simulink model "sim_config2a"  (R2023b)
settings: Solver=ode4  StartTime=0.0  StopTime=60  FixedStep=0.01  RelTol=1e-3
undefined symbols (not defined in the file): aircraft, alt_ground, atmosphere, envir, g, pos_ref, struct2cell, u0, wind
libraries: unit_conversions_lib x19, flightgear_visualization_lib x2, joystick_lib x1, atmosphere_lib x1, axes_transformation_lib x1, syntrac_lib x1
settings Model: Creator=yannic  LastModifiedBy=Ole Bunde

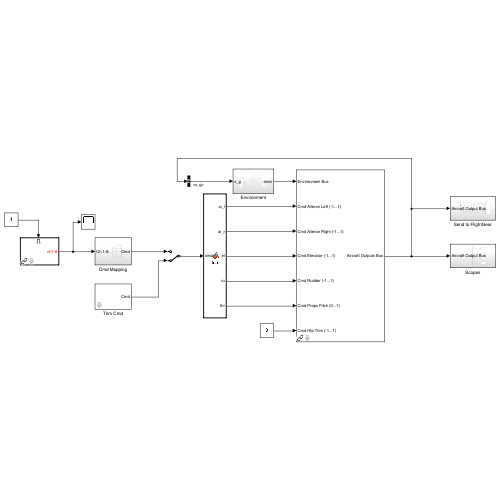
[thumbnail: Simulink's stored preview of the top-level diagram]
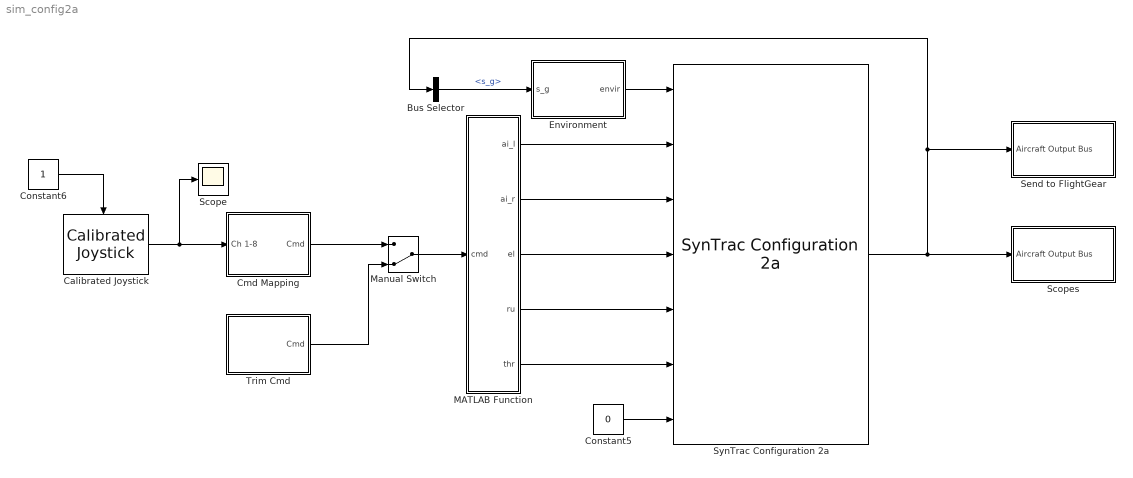
== system sim_config2a ==
  Bus Selector : BusSelector  OutputSignals=rigidBodyBus.s_g
  Calibrated Joystick : joystick_lib/Calibrated Joystick  jystck=jystck  joyid=1
      settings: SourceProductName=LADAC
  Cmd Mapping : Subsystem
  Constant5 : Constant  Value=0
  Constant6 : Constant
  Environment : Subsystem
  MATLAB Function : MATLAB Function  TreatAsAtomicUnit=on
  Manual Switch : ManualSwitch  CurrentSetting=0
  Scope : Scope
  Scopes : Subsystem
  Send to FlightGear : Subsystem
  SynTrac Configuration 2a : syntrac_lib/SynTrac Configuration 2a  aircraft=aircraft  ic=ic
  Trim Cmd : Subsystem  mask{num_props=length(aircraft.prop)}
      mask prompts: num_props "Number of Propellers"
  wires:
  Environment/1(envir) -> SynTrac Configuration 2a/1
  SynTrac Configuration 2a/1 -> Send to FlightGear/1(Aircraft Output Bus), Bus Selector/1, Scopes/1(Aircraft Output Bus)
  Bus Selector/1 -> Environment/1(s_g)  "<s_g>"
  Constant5/1 -> SynTrac Configuration 2a/7
  Constant6/1 -> Calibrated Joystick/Enable
  Calibrated Joystick/1 -> Cmd Mapping/1(Ch 1-8), Scope/1
  Cmd Mapping/1(Cmd) -> Manual Switch/1
  Manual Switch/1 -> MATLAB Function/1(cmd)
  MATLAB Function/5(thr) -> SynTrac Configuration 2a/6
  MATLAB Function/4(ru) -> SynTrac Configuration 2a/5
  MATLAB Function/2(ai_r) -> SynTrac Configuration 2a/3
  MATLAB Function/1(ai_l) -> SynTrac Configuration 2a/2
  Trim Cmd/1(Cmd) -> Manual Switch/2
  MATLAB Function/3(el) -> SynTrac Configuration 2a/4

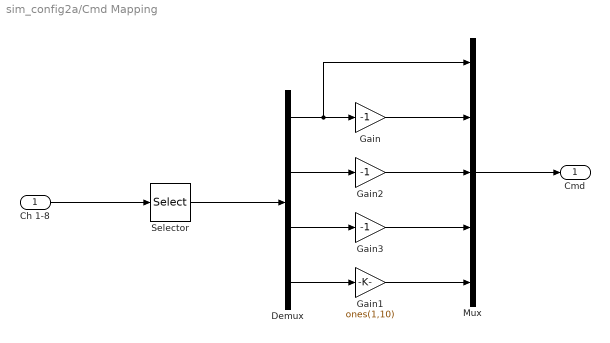
== system sim_config2a/Cmd Mapping ==
  Ch 1-8 : Inport
  Demux : Demux
  Gain : Gain  Gain=-1
  Gain1 : Gain  Gain=ones(1,10)
  Gain2 : Gain  Gain=-1
  Gain3 : Gain  Gain=-1
  Mux : Mux  Inputs=5
  Selector : Selector  InputPortWidth=8  IndexOptions=Index vector (dialog)  Indices=[1,2,3,4]  OutputSizes=1
  Cmd : Outport
  wires:
  Gain1/1 -> Mux/5
  Demux/4 -> Gain1/1
  Gain/1 -> Mux/2
  Gain2/1 -> Mux/3
  Demux/3 -> Gain3/1
  Demux/2 -> Gain2/1
  Demux/1 -> Mux/1, Gain/1
  Ch 1-8/1 -> Selector/1
  Gain3/1 -> Mux/4
  Mux/1 -> Cmd/1
  Selector/1 -> Demux/1

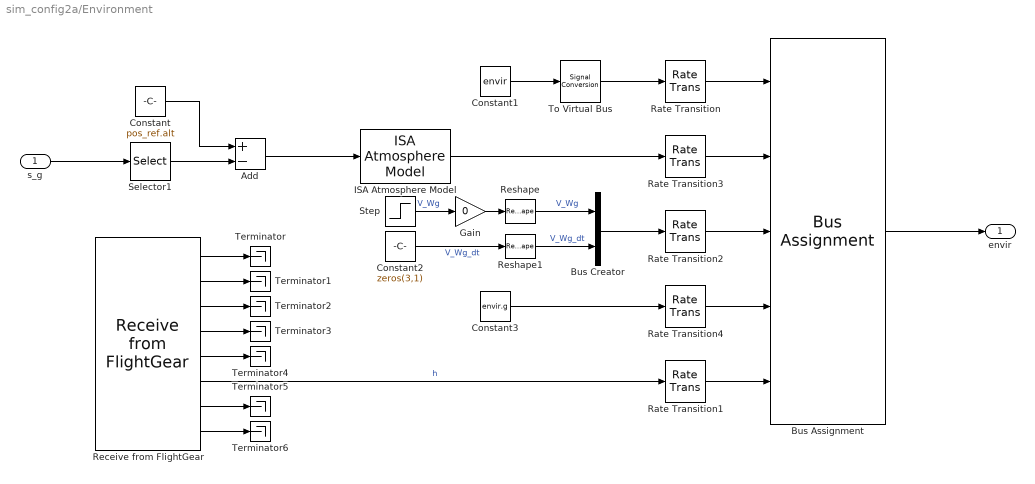
== system sim_config2a/Environment ==
  s_g : Inport
  Add : Sum  Inputs=+-
  Bus Assignment : BusAssignment  AssignedSignals=atmosphere,wind,g,alt_ground
  Bus Creator : BusCreator  Inputs=2
  Constant : Constant  Value=pos_ref.alt
  Constant1 : Constant  Value=envir  OutDataTypeStr=Bus: envirBus
  Constant2 : Constant  Value=zeros(3,1)
  Constant3 : Constant  Value=envir.g
  Gain : Gain  Gain=0
  ISA Atmosphere Model : atmosphere_lib/ISA Atmosphere Model
      settings: SourceProductName=LADAC
  Rate Transition{,1..4} (5 alike) : RateTransition
  Receive from FlightGear : flightgear_visualization_lib/Receive from FlightGear  ip_address='127.0.0.1'  ip_port=5503  sample_time=1/20  blocking_time=0  is_aerocntrl=off  is_engine=off  is_fuel=off  is_land=off  is_avionics=off  is_envir=on
  Reshape : Reshape  OutputDimensionality=Column vector (2-D)
  Reshape1 : Reshape  OutputDimensionality=Column vector (2-D)
  Selector1 : Selector  InputPortWidth=3  IndexOptions=Index vector (dialog)  Indices=3  OutputSizes=1
  Step : Step  Time=3  After=[0;9;0]  SampleTime=0
  Terminator{,1..6} (7 alike) : Terminator
  To Virtual Bus : SignalConversion  ConversionOutput=Virtual bus  OverrideOpt=off
  envir : Outport  VectorParamsAs1DForOutWhenUnconnected=off
  wires:
  Rate Transition2/1 -> Bus Assignment/3
  Rate Transition3/1 -> Bus Assignment/2
  Bus Assignment/1 -> envir/1
  Rate Transition/1 -> Bus Assignment/1
  ISA Atmosphere Model/1 -> Rate Transition3/1
  Step/1 -> Gain/1  "V_Wg"
  Rate Transition1/1 -> Bus Assignment/5
  Constant1/1 -> To Virtual Bus/1
  s_g/1 -> Selector1/1
  Bus Creator/1 -> Rate Transition2/1
  Constant2/1 -> Reshape1/1  "V_Wg_dt"
  Rate Transition4/1 -> Bus Assignment/4
  Constant3/1 -> Rate Transition4/1
  Gain/1 -> Reshape/1
  Constant/1 -> Add/1
  Add/1 -> ISA Atmosphere Model/1
  Selector1/1 -> Add/2
  To Virtual Bus/1 -> Rate Transition/1
  Reshape/1 -> Bus Creator/1  "V_Wg"
  Reshape1/1 -> Bus Creator/2  "V_Wg_dt"
  Receive from FlightGear/3 -> Terminator2/1
  Receive from FlightGear/1 -> Terminator/1
  Receive from FlightGear/6 -> Rate Transition1/1  "h"
  Receive from FlightGear/2 -> Terminator1/1
  Receive from FlightGear/5 -> Terminator4/1
  Receive from FlightGear/7 -> Terminator5/1
  Receive from FlightGear/4 -> Terminator3/1
  Receive from FlightGear/8 -> Terminator6/1

== system sim_config2a/Scopes ==
  Aircraft Output Bus : Inport
  Actuators : Subsystem
  Aerodynamics : Subsystem
  Bus Selector : BusSelector  OutputSignals=rigidBodyBus,aeroBus,actuatorsBus,propBus
  Propellers : Subsystem
  Rigid Body : Subsystem
  wires:
  Aircraft Output Bus/1 -> Bus Selector/1
  Bus Selector/1 -> Rigid Body/1(rigidBodyBus)  "<rigidBodyBus>"
  Bus Selector/3 -> Actuators/1(actuatorsBus)  "<actuatorsBus>"
  Bus Selector/2 -> Aerodynamics/1(aeroBus)  "<aeroBus>"
  Bus Selector/4 -> Propellers/1(propBus)  "<propBus>"

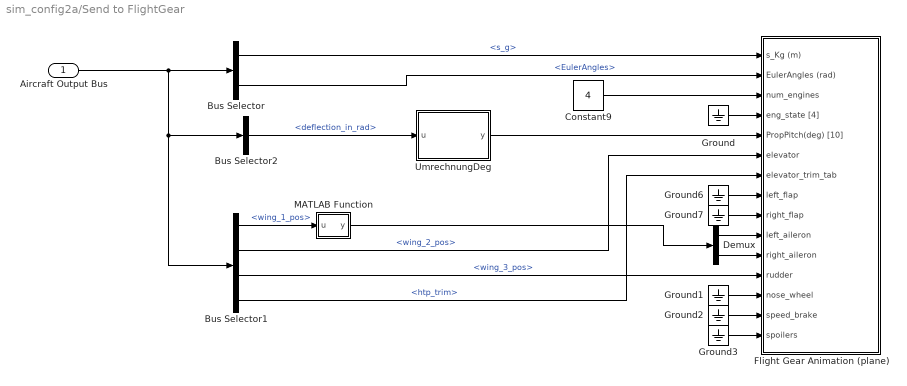
== system sim_config2a/Send to FlightGear ==
  Aircraft Output Bus : Inport
  Bus Selector : BusSelector  OutputSignals=rigidBodyBus.s_g,rigidBodyBus.EulerAngles
  Bus Selector1 : BusSelector  OutputSignals=actuatorsBus.wing_1_pos,actuatorsBus.wing_2_pos,actuatorsBus.wing_3_pos,actuatorsBus.htp_trim
  Bus Selector2 : BusSelector  OutputSignals=actuatorsBus.props_pitch.deflection_in_rad
  Constant9 : Constant  Value=4
  Demux : Demux  Outputs=2
  Flight Gear Animation (plane) : Subsystem  AncestorBlock=flightgear_visualization_lib/Flight Gear Animation (plane)  mask{inital_lat=pos_ref.lat, inital_long=pos_ref.lon, inital_height=pos_ref.alt, remoteURL='127.0.0.1', remotePort=5502}
      mask prompts: inital_lat "Inital Latitude (deg)"; inital_long "Inital Longitude (deg)"; inital_height "Inital Height (m)"; remoteURL "URL of FlightGear, e.g. '127.0.0.1'"; remotePort "Port of FlightGear, e.g. 5502"
      mask TypeOptions remoteURL: Send to FlightGear/remoteURL
      mask TypeOptions remotePort: Send to FlightGear/remotePort
      mask DialogControl GroupDesc Prompt: Initial Latitude
  Ground{,1..3,6..7} (6 alike) : Ground
  MATLAB Function : MATLAB Function  TreatAsAtomicUnit=on
  UmrechnungDeg : MATLAB Function  TreatAsAtomicUnit=on
  wires:
  Bus Selector/1 -> Flight Gear Animation (plane)/1(s_Kg (m))  "<s_g>"
  Bus Selector/2 -> Flight Gear Animation (plane)/2(EulerAngles (rad))  "<EulerAngles>"
  Constant9/1 -> Flight Gear Animation (plane)/3(num_engines)
  Ground/1 -> Flight Gear Animation (plane)/4(eng_state [4])
  Ground1/1 -> Flight Gear Animation (plane)/13(nose_wheel)
  Ground2/1 -> Flight Gear Animation (plane)/14(speed_brake)
  Ground3/1 -> Flight Gear Animation (plane)/15(spoilers)
  Aircraft Output Bus/1 -> Bus Selector1/1, Bus Selector2/1, Bus Selector/1
  Bus Selector1/2 -> Flight Gear Animation (plane)/6(elevator)  "<wing_2_pos>"
  Bus Selector1/4 -> Flight Gear Animation (plane)/7(elevator_trim_tab)  "<htp_trim>"
  Ground6/1 -> Flight Gear Animation (plane)/8(left_flap)
  Ground7/1 -> Flight Gear Animation (plane)/9(right_flap)
  Bus Selector1/3 -> Flight Gear Animation (plane)/12(rudder)  "<wing_3_pos>"
  Bus Selector1/1 -> MATLAB Function/1(u)  "<wing_1_pos>"
  Demux/1 -> Flight Gear Animation (plane)/10(left_aileron)
  Demux/2 -> Flight Gear Animation (plane)/11(right_aileron)
  MATLAB Function/1(y) -> Demux/1
  Bus Selector2/1 -> UmrechnungDeg/1(u)  "<deflection_in_rad>"
  UmrechnungDeg/1(y) -> Flight Gear Animation (plane)/5(PropPitch(deg) [10])

== system sim_config2a/Trim Cmd ==
  u0 : Constant  Value=cell2mat(struct2cell(u0))
  u0 to Cmd : MATLAB Function  TreatAsAtomicUnit=on
  Cmd : Outport
  wires:
  u0/1 -> u0 to Cmd/1(u0)
  u0 to Cmd/1(cmd) -> Cmd/1

== system sim_config2a/Scopes/Actuators ==
  actuatorsBus : Inport
  Aileron Deflections (deg) (Downward Positive) : Scope
  Bus Selector : BusSelector  OutputSignals=wing_1_pos,wing_2_pos,wing_3_pos,props_pitch.deflection_in_rad,htp_trim
  Elevator Deflection (deg) (Downward Positive) : Scope
  Propeller Pitch (deg) : Scope
  Rudder Deflection (deg) (Right Positive) : Scope
  Scope : Scope
  rad2deg : unit_conversions_lib/rad2deg
      settings: SourceProductName=LADAC
  wires:
  actuatorsBus/1 -> Bus Selector/1
  Bus Selector/1 -> Aileron Deflections (deg) (Downward Positive)/1  "<wing_1_pos>"
  Bus Selector/2 -> Elevator Deflection (deg) (Downward Positive)/1  "<wing_2_pos>"
  Bus Selector/3 -> Rudder Deflection (deg) (Right Positive)/1  "<wing_3_pos>"
  Bus Selector/4 -> rad2deg/1  "<deflection_in_rad>"
  rad2deg/1 -> Propeller Pitch (deg)/1
  Bus Selector/5 -> Scope/1  "<htp_trim>"

== system sim_config2a/Scopes/Aerodynamics ==
  aeroBus : Inport
  Bus Selector : BusSelector  OutputSignals=main,htp,vtp,R_Ab,Q_Ab
  Force Vector (N) (Body Frame) : Scope
  Horizontal Tailplane : Subsystem
  Main Wing : Subsystem
  Moment Vector (Nm) (Body Frame) : Scope
  Vertical Tailplane : Subsystem
  wires:
  aeroBus/1 -> Bus Selector/1
  Bus Selector/1 -> Main Wing/1(wingBus)  "<main>"
  Bus Selector/2 -> Horizontal Tailplane/1(wingBus)  "<htp>"
  Bus Selector/3 -> Vertical Tailplane/1(wingBus)  "<vtp>"
  Bus Selector/4 -> Force Vector (N) (Body Frame)/1  "<R_Ab>"
  Bus Selector/5 -> Moment Vector (Nm) (Body Frame)/1  "<Q_Ab>"

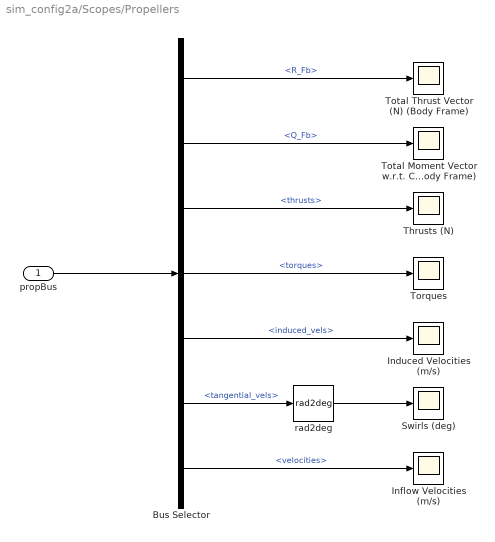
== system sim_config2a/Scopes/Propellers ==
  propBus : Inport
  Bus Selector : BusSelector  OutputSignals=R_Fb,Q_Fb,thrusts,torques,induced_vels,tangential_vels,velocities
  Induced Velocities (m/s) : Scope
  Inflow Velocities (m/s) : Scope
  Swirls (deg) : Scope
  Thrusts (N) : Scope
  Torques : Scope
  Total Moment Vector w.r.t. CG (Nm) (Body Frame) : Scope
  Total Thrust Vector (N) (Body Frame) : Scope
  rad2deg : unit_conversions_lib/rad2deg
      settings: SourceProductName=LADAC
  wires:
  propBus/1 -> Bus Selector/1
  Bus Selector/1 -> Total Thrust Vector (N) (Body Frame)/1  "<R_Fb>"
  Bus Selector/2 -> Total Moment Vector w.r.t. CG (Nm) (Body Frame)/1  "<Q_Fb>"
  Bus Selector/3 -> Thrusts (N)/1  "<thrusts>"
  Bus Selector/4 -> Torques/1  "<torques>"
  Bus Selector/5 -> Induced Velocities (m/s)/1  "<induced_vels>"
  Bus Selector/6 -> rad2deg/1  "<tangential_vels>"
  rad2deg/1 -> Swirls (deg)/1
  Bus Selector/7 -> Inflow Velocities (m/s)/1  "<velocities>"

== system sim_config2a/Scopes/Rigid Body ==
  rigidBodyBus : Inport
  Angular Rates (deg/s) : Scope
  Bus Selector : BusSelector  OutputSignals=omega_Kb,EulerAngles,s_g,V_Kg,V_Kb
  Euler Angles (deg) : Scope
  Position (m) : Scope
  Velocity FRD (m/s) : Scope
  Velocity NED (m/s) : Scope
  rad2deg : unit_conversions_lib/rad2deg
      settings: SourceProductName=LADAC
  rad2deg1 : unit_conversions_lib/rad2deg
      settings: SourceProductName=LADAC
  wires:
  rigidBodyBus/1 -> Bus Selector/1
  Bus Selector/1 -> rad2deg/1  "<omega_Kb>"
  rad2deg/1 -> Angular Rates (deg/s)/1
  Bus Selector/2 -> rad2deg1/1  "<EulerAngles>"
  rad2deg1/1 -> Euler Angles (deg)/1
  Bus Selector/3 -> Position (m)/1  "<s_g>"
  Bus Selector/4 -> Velocity NED (m/s)/1  "<V_Kg>"
  Bus Selector/5 -> Velocity FRD (m/s)/1  "<V_Kb>"

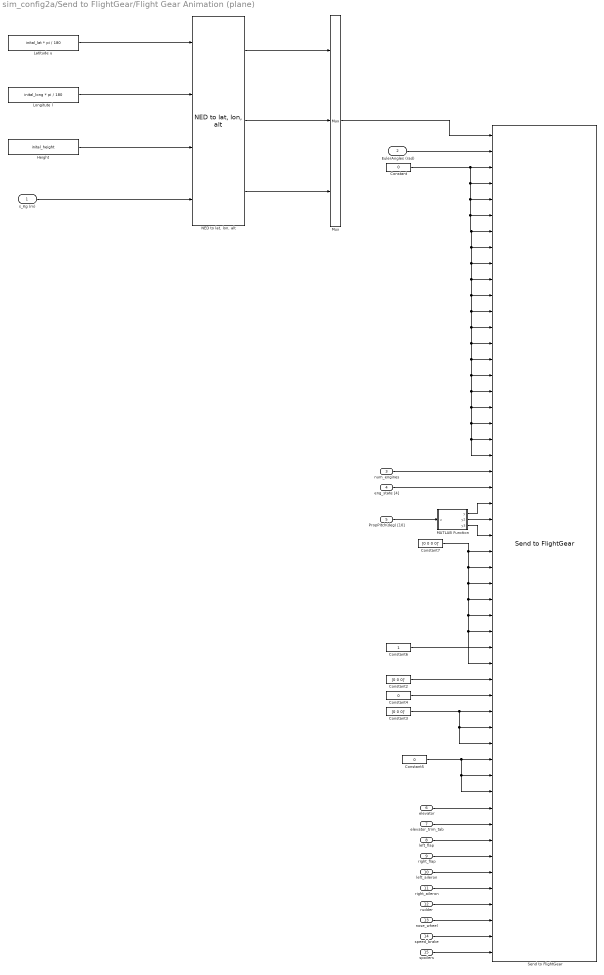
== system sim_config2a/Send to FlightGear/Flight Gear Animation (plane) ==
  s_Kg (m) : Inport
  EulerAngles (rad) : Inport  Port=2
  num_engines : Inport  Port=3  PortDimensions=[1]
  eng_state [4] : Inport  Port=4  PortDimensions=[4]
  PropPitch(deg) [10] : Inport  Port=5  PortDimensions=[10]
  elevator : Inport  Port=6  PortDimensions=[1]
  elevator_trim_tab : Inport  Port=7  PortDimensions=[1]
  left_flap : Inport  Port=8  PortDimensions=[1]
  right_flap : Inport  Port=9  PortDimensions=[1]
  left_aileron : Inport  Port=10  PortDimensions=[1]
  right_aileron : Inport  Port=11  PortDimensions=[1]
  rudder : Inport  Port=12  PortDimensions=[1]
  nose_wheel : Inport  Port=13  PortDimensions=[1]
  speed_brake : Inport  Port=14  PortDimensions=[1]
  spoilers : Inport  Port=15  PortDimensions=[1]
  Constant : Constant  Value=0
  Constant2 : Constant  Value=[0 0 0]'  VectorParams1D=off
  Constant3 : Constant  Value=[0 0 0]'  VectorParams1D=off
  Constant4 : Constant  Value=0
  Constant5 : Constant  Value=0
  Constant6 : Constant
  Constant7 : Constant  Value=[0 0 0 0]'  VectorParams1D=off
  Height : Constant  Value=inital_height
  Latitude u : Constant  Value=inital_lat * pi / 180
  Longitute l : Constant  Value=inital_long * pi / 180
  MATLAB Function : MATLAB Function  TreatAsAtomicUnit=on
  Mux : Mux  Inputs=3
  "NED to lat, lon, alt" : axes_transformation_lib/NED to lat, lon, alt  SystemSampleTime=-1  VariantActivationTime=update diagram  AllowFlexibleInterface=on  Latency=0  AutoFrameSizeCalculation=off
      settings: SourceProductName=LADAC
  Send to FlightGear : flightgear_visualization_lib/Send to FlightGear  remotePort=remotePort  remoteURL=remoteURL
  wires:
  Constant6/1 -> Send to FlightGear/33
  Constant5/1 -> Send to FlightGear/41, Send to FlightGear/42, Send to FlightGear/40
  Constant4/1 -> Send to FlightGear/36
  Constant3/1 -> Send to FlightGear/38, Send to FlightGear/39, Send to FlightGear/37
  Constant2/1 -> Send to FlightGear/35
  Constant7/1 -> Send to FlightGear/34, Send to FlightGear/32, Send to FlightGear/31, Send to FlightGear/30, Send to FlightGear/29, Send to FlightGear/28, Send to FlightGear/27
  Constant/1 -> Send to FlightGear/20, Send to FlightGear/21, Send to FlightGear/19, Send to FlightGear/18, Send to FlightGear/17, Send to FlightGear/16, Send to FlightGear/15, Send to FlightGear/14, Send to FlightGear/13, Send to FlightGear/12, Send to FlightGear/11, Send to FlightGear/10, Send to FlightGear/9, Send to FlightGear/8, Send to FlightGear/7, Send to FlightGear/6, Send to FlightGear/5, Send to FlightGear/4, Send to FlightGear/3
  PropPitch(deg) [10]/1 -> MATLAB Function/1(u)
  eng_state [4]/1 -> Send to FlightGear/23
  num_engines/1 -> Send to FlightGear/22
  right_aileron/1 -> Send to FlightGear/48
  left_aileron/1 -> Send to FlightGear/47
  right_flap/1 -> Send to FlightGear/46
  left_flap/1 -> Send to FlightGear/45
  elevator_trim_tab/1 -> Send to FlightGear/44
  elevator/1 -> Send to FlightGear/43
  rudder/1 -> Send to FlightGear/49
  nose_wheel/1 -> Send to FlightGear/50
  speed_brake/1 -> Send to FlightGear/51
  spoilers/1 -> Send to FlightGear/52
  s_Kg (m)/1 -> "NED to lat, lon, alt"/4
  EulerAngles (rad)/1 -> Send to FlightGear/2
  Latitude u/1 -> "NED to lat, lon, alt"/1
  Longitute l/1 -> "NED to lat, lon, alt"/2
  Height/1 -> "NED to lat, lon, alt"/3
  "NED to lat, lon, alt"/3 -> Mux/3
  "NED to lat, lon, alt"/2 -> Mux/2
  "NED to lat, lon, alt"/1 -> Mux/1
  Mux/1 -> Send to FlightGear/1
  MATLAB Function/1(y) -> Send to FlightGear/24
  MATLAB Function/2(y2) -> Send to FlightGear/25
  MATLAB Function/3(y3) -> Send to FlightGear/26

== system sim_config2a/Scopes/Aerodynamics/Horizontal Tailplane ==
  wingBus : Inport
  Aerodynamics : Subsystem
  Body : Subsystem
  Bus Selector : BusSelector  OutputSignals=body,aero,external.V_Wb
  Wind/Slipstream : Subsystem
  wires:
  Bus Selector/3 -> Wind/Slipstream/1(V_Wb)  "<V_Wb>"
  Bus Selector/2 -> Aerodynamics/1(aeroBus)  "<aero>"
  Bus Selector/1 -> Body/1(bodyBus)  "<body>"
  wingBus/1 -> Bus Selector/1

== system sim_config2a/Scopes/Aerodynamics/Main Wing ==
  wingBus : Inport
  Aerodynamics : Subsystem
  Body : Subsystem
  Bus Selector : BusSelector  OutputSignals=body,aero,external.V_Wb
  Wind/Slipstream : Subsystem
  wires:
  wingBus/1 -> Bus Selector/1
  Bus Selector/1 -> Body/1(bodyBus)  "<body>"
  Bus Selector/2 -> Aerodynamics/1(aeroBus)  "<aero>"
  Bus Selector/3 -> Wind/Slipstream/1(V_Wb)  "<V_Wb>"

== system sim_config2a/Scopes/Aerodynamics/Vertical Tailplane ==
  wingBus : Inport
  Aerodynamics : Subsystem
  Body : Subsystem
  Bus Selector : BusSelector  OutputSignals=body,aero,external.V_Wb
  Wind/Slipstream : Subsystem
  wires:
  wingBus/1 -> Bus Selector/1
  Bus Selector/1 -> Body/1(bodyBus)  "<body>"
  Bus Selector/2 -> Aerodynamics/1(aeroBus)  "<aero>"
  Bus Selector/3 -> Wind/Slipstream/1(V_Wb)  "<V_Wb>"

== system sim_config2a/Scopes/Aerodynamics/Horizontal Tailplane/Aerodynamics ==
  aeroBus : Inport
  Bus Selector : BusSelector  OutputSignals=circulation,coeff_loc,coeff_glob,force_loc,force_glob,local_inflow
  Circulation : Subsystem
  Global Coefficients : Subsystem
  Global Forces : Subsystem
  Local Coefficients : Subsystem
  Local Forces : Subsystem
  Local Inflow : Subsystem
  wires:
  Bus Selector/6 -> Local Inflow/1(localInflowBus)  "<local_inflow>"
  Bus Selector/5 -> Global Forces/1(forceGlobBus)  "<force_glob>"
  Bus Selector/4 -> Local Forces/1(forceLocBus)  "<force_loc>"
  Bus Selector/3 -> Global Coefficients/1(coeffGlobBus)  "<coeff_glob>"
  aeroBus/1 -> Bus Selector/1
  Bus Selector/1 -> Circulation/1(circulationBus)  "<circulation>"
  Bus Selector/2 -> Local Coefficients/1(coeffLocBus)  "<coeff_loc>"

== system sim_config2a/Scopes/Aerodynamics/Horizontal Tailplane/Body ==
  bodyBus : Inport
  Airspeed (m/s) : Scope
  Angle of Attack (deg) : Scope
  Bus Selector : BusSelector  OutputSignals=V,alpha,beta
  Sideslip Angle (deg) : Scope
  rad2deg : unit_conversions_lib/rad2deg
      settings: SourceProductName=LADAC
  rad2deg1 : unit_conversions_lib/rad2deg
      settings: SourceProductName=LADAC
  wires:
  rad2deg1/1 -> Sideslip Angle (deg)/1
  Bus Selector/3 -> rad2deg1/1  "<beta>"
  rad2deg/1 -> Angle of Attack (deg)/1
  Bus Selector/2 -> rad2deg/1  "<alpha>"
  Bus Selector/1 -> Airspeed (m/s)/1  "<V>"
  bodyBus/1 -> Bus Selector/1

== system sim_config2a/Scopes/Aerodynamics/Horizontal Tailplane/Wind//Slipstream ==
  V_Wb : Inport
  Demux : MATLAB Function  TreatAsAtomicUnit=on
  Downward Wind/Slipstream Velocities (m/s) (Body Frame) : Scope
  Forward Wind/Slipstream Velocities (m/s) (Body Frame) : Scope
  Lateral Wind/Slipstream Velocities (m/s) (Body Frame) : Scope
  wires:
  Demux/3(z) -> Downward Wind/Slipstream Velocities (m/s) (Body Frame)/1  "w_Wb"
  Demux/2(y) -> Lateral Wind/Slipstream Velocities (m/s) (Body Frame)/1  "v_Wb"
  Demux/1(x) -> Forward Wind/Slipstream Velocities (m/s) (Body Frame)/1  "u_Wb"
  V_Wb/1 -> Demux/1(xyz)

== system sim_config2a/Scopes/Aerodynamics/Main Wing/Aerodynamics ==
  aeroBus : Inport
  Bus Selector : BusSelector  OutputSignals=circulation,coeff_loc,coeff_glob,force_loc,force_glob,local_inflow
  Circulation : Subsystem
  Global Coefficients : Subsystem
  Global Forces : Subsystem
  Local Coefficients : Subsystem
  Local Forces : Subsystem
  Local Inflow : Subsystem
  wires:
  Bus Selector/2 -> Local Coefficients/1(coeffLocBus)  "<coeff_loc>"
  Bus Selector/1 -> Circulation/1(circulationBus)  "<circulation>"
  aeroBus/1 -> Bus Selector/1
  Bus Selector/3 -> Global Coefficients/1(coeffGlobBus)  "<coeff_glob>"
  Bus Selector/4 -> Local Forces/1(forceLocBus)  "<force_loc>"
  Bus Selector/5 -> Global Forces/1(forceGlobBus)  "<force_glob>"
  Bus Selector/6 -> Local Inflow/1(localInflowBus)  "<local_inflow>"

== system sim_config2a/Scopes/Aerodynamics/Main Wing/Body ==
  bodyBus : Inport
  Airspeed (m/s) : Scope
  Angle of Attack (deg) : Scope
  Bus Selector : BusSelector  OutputSignals=V,alpha,beta
  Sideslip Angle (deg) : Scope
  rad2deg : unit_conversions_lib/rad2deg
      settings: SourceProductName=LADAC
  rad2deg1 : unit_conversions_lib/rad2deg
      settings: SourceProductName=LADAC
  wires:
  bodyBus/1 -> Bus Selector/1
  Bus Selector/1 -> Airspeed (m/s)/1  "<V>"
  Bus Selector/2 -> rad2deg/1  "<alpha>"
  rad2deg/1 -> Angle of Attack (deg)/1
  Bus Selector/3 -> rad2deg1/1  "<beta>"
  rad2deg1/1 -> Sideslip Angle (deg)/1

== system sim_config2a/Scopes/Aerodynamics/Main Wing/Wind//Slipstream ==
  V_Wb : Inport
  Demux : MATLAB Function  TreatAsAtomicUnit=on
  Downward Wind/Slipstream Velocities (m/s) (Body Frame) : Scope
  Forward Wind/Slipstream Velocities (m/s) (Body Frame) : Scope
  Lateral Wind/Slipstream Velocities (m/s) (Body Frame) : Scope
  wires:
  V_Wb/1 -> Demux/1(xyz)
  Demux/1(x) -> Forward Wind/Slipstream Velocities (m/s) (Body Frame)/1  "u_Wb"
  Demux/2(y) -> Lateral Wind/Slipstream Velocities (m/s) (Body Frame)/1  "v_Wb"
  Demux/3(z) -> Downward Wind/Slipstream Velocities (m/s) (Body Frame)/1  "w_Wb"

== system sim_config2a/Scopes/Aerodynamics/Vertical Tailplane/Aerodynamics ==
  aeroBus : Inport
  Bus Selector : BusSelector  OutputSignals=circulation,coeff_loc,coeff_glob,force_loc,force_glob,local_inflow
  Circulation : Subsystem
  Global Coefficients : Subsystem
  Global Forces : Subsystem
  Local Coefficients : Subsystem
  Local Forces : Subsystem
  Local Inflow : Subsystem
  wires:
  Bus Selector/2 -> Local Coefficients/1(coeffLocBus)  "<coeff_loc>"
  Bus Selector/1 -> Circulation/1(circulationBus)  "<circulation>"
  aeroBus/1 -> Bus Selector/1
  Bus Selector/3 -> Global Coefficients/1(coeffGlobBus)  "<coeff_glob>"
  Bus Selector/4 -> Local Forces/1(forceLocBus)  "<force_loc>"
  Bus Selector/5 -> Global Forces/1(forceGlobBus)  "<force_glob>"
  Bus Selector/6 -> Local Inflow/1(localInflowBus)  "<local_inflow>"

== system sim_config2a/Scopes/Aerodynamics/Vertical Tailplane/Body ==
  bodyBus : Inport
  Airspeed (m/s) : Scope
  Angle of Attack (deg) : Scope
  Bus Selector : BusSelector  OutputSignals=V,alpha,beta
  Sideslip Angle (deg) : Scope
  rad2deg : unit_conversions_lib/rad2deg
      settings: SourceProductName=LADAC
  rad2deg1 : unit_conversions_lib/rad2deg
      settings: SourceProductName=LADAC
  wires:
  bodyBus/1 -> Bus Selector/1
  Bus Selector/1 -> Airspeed (m/s)/1  "<V>"
  Bus Selector/2 -> rad2deg/1  "<alpha>"
  rad2deg/1 -> Angle of Attack (deg)/1
  Bus Selector/3 -> rad2deg1/1  "<beta>"
  rad2deg1/1 -> Sideslip Angle (deg)/1

== system sim_config2a/Scopes/Aerodynamics/Vertical Tailplane/Wind//Slipstream ==
  V_Wb : Inport
  Demux : MATLAB Function  TreatAsAtomicUnit=on
  Downward Wind/Slipstream Velocities (m/s) (Body Frame) : Scope
  Forward Wind/Slipstream Velocities (m/s) (Body Frame) : Scope
  Lateral Wind/Slipstream Velocities (m/s) (Body Frame) : Scope
  wires:
  V_Wb/1 -> Demux/1(xyz)
  Demux/1(x) -> Forward Wind/Slipstream Velocities (m/s) (Body Frame)/1  "u_Wb"
  Demux/2(y) -> Lateral Wind/Slipstream Velocities (m/s) (Body Frame)/1  "v_Wb"
  Demux/3(z) -> Downward Wind/Slipstream Velocities (m/s) (Body Frame)/1  "w_Wb"

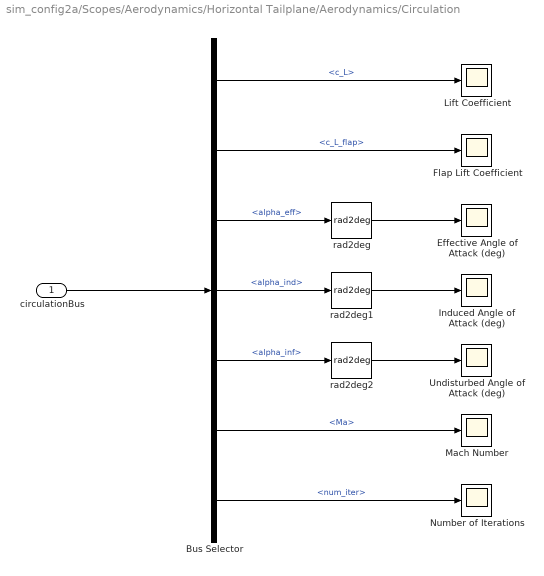
== system sim_config2a/Scopes/Aerodynamics/Horizontal Tailplane/Aerodynamics/Circulation ==
  circulationBus : Inport
  Bus Selector : BusSelector  OutputSignals=c_L,c_L_flap,alpha_eff,alpha_ind,alpha_inf,Ma,num_iter
  Effective Angle of Attack (deg) : Scope
  Flap Lift Coefficient : Scope
  Induced Angle of Attack (deg) : Scope
  Lift Coefficient : Scope
  Mach Number : Scope
  Number of Iterations : Scope
  Undisturbed Angle of Attack (deg) : Scope
  rad2deg : unit_conversions_lib/rad2deg
      settings: SourceProductName=LADAC
  rad2deg1 : unit_conversions_lib/rad2deg
      settings: SourceProductName=LADAC
  rad2deg2 : unit_conversions_lib/rad2deg
      settings: SourceProductName=LADAC
  wires:
  Bus Selector/7 -> Number of Iterations/1  "<num_iter>"
  Bus Selector/6 -> Mach Number/1  "<Ma>"
  rad2deg2/1 -> Undisturbed Angle of Attack (deg)/1
  Bus Selector/5 -> rad2deg2/1  "<alpha_inf>"
  rad2deg1/1 -> Induced Angle of Attack (deg)/1
  Bus Selector/4 -> rad2deg1/1  "<alpha_ind>"
  rad2deg/1 -> Effective Angle of Attack (deg)/1
  Bus Selector/3 -> rad2deg/1  "<alpha_eff>"
  Bus Selector/2 -> Flap Lift Coefficient/1  "<c_L_flap>"
  Bus Selector/1 -> Lift Coefficient/1  "<c_L>"
  circulationBus/1 -> Bus Selector/1

== system sim_config2a/Scopes/Aerodynamics/Horizontal Tailplane/Aerodynamics/Global Coefficients ==
  coeffGlobBus : Inport
  Bus Selector : BusSelector  OutputSignals=C_XYZ_b,C_lmn_b
  Force Coefficients (Body Frame) : Scope
  Moment Coefficients (Body Frame) : Scope
  wires:
  Bus Selector/2 -> Moment Coefficients (Body Frame)/1  "<C_lmn_b>"
  Bus Selector/1 -> Force Coefficients (Body Frame)/1  "<C_XYZ_b>"
  coeffGlobBus/1 -> Bus Selector/1

== system sim_config2a/Scopes/Aerodynamics/Horizontal Tailplane/Aerodynamics/Global Forces ==
  forceGlobBus : Inport
  Bus Selector : BusSelector  OutputSignals=R_b,Q_origin_b
  Force Vector (N) (Body Frame) : Scope
  Moment Vector w.r.t. CG (N) (Body Frame) : Scope
  wires:
  Bus Selector/2 -> Moment Vector w.r.t. CG (N) (Body Frame)/1  "<Q_origin_b>"
  Bus Selector/1 -> Force Vector (N) (Body Frame)/1  "<R_b>"
  forceGlobBus/1 -> Bus Selector/1

== system sim_config2a/Scopes/Aerodynamics/Horizontal Tailplane/Aerodynamics/Local Coefficients ==
  coeffLocBus : Inport
  Bus Selector : BusSelector  OutputSignals=c_XYZ_b,c_m_airfoil
  Demux : MATLAB Function  TreatAsAtomicUnit=on
  Downward Force Coefficient (Body Frame) : Scope
  Forward Force Coefficient (Body Frame) : Scope
  Lateral Force Coefficient (Body Frame) : Scope
  Pitching Moment Coefficient (c/4) : Scope
  wires:
  Bus Selector/2 -> Pitching Moment Coefficient (c/4)/1  "<c_m_airfoil>"
  Demux/3(z) -> Downward Force Coefficient (Body Frame)/1  "c_Zb"
  Demux/2(y) -> Lateral Force Coefficient (Body Frame)/1  "c_Yb"
  Demux/1(x) -> Forward Force Coefficient (Body Frame)/1  "c_Xb"
  Bus Selector/1 -> Demux/1(xyz)  "<c_XYZ_b>"
  coeffLocBus/1 -> Bus Selector/1

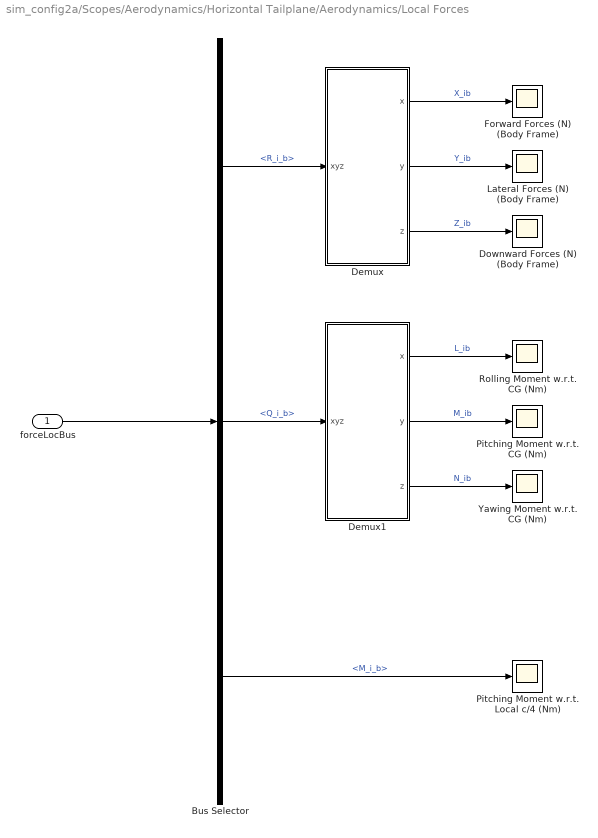
== system sim_config2a/Scopes/Aerodynamics/Horizontal Tailplane/Aerodynamics/Local Forces ==
  forceLocBus : Inport
  Bus Selector : BusSelector  OutputSignals=R_i_b,Q_i_b,M_i_b
  Demux : MATLAB Function  TreatAsAtomicUnit=on
  Demux1 : MATLAB Function  TreatAsAtomicUnit=on
  Downward Forces (N) (Body Frame) : Scope
  Forward Forces (N) (Body Frame) : Scope
  Lateral Forces (N) (Body Frame) : Scope
  Pitching Moment w.r.t. CG (Nm) : Scope
  Pitching Moment w.r.t. Local c/4 (Nm) : Scope
  Rolling Moment w.r.t. CG (Nm) : Scope
  Yawing Moment w.r.t. CG (Nm) : Scope
  wires:
  Bus Selector/3 -> Pitching Moment w.r.t. Local c/4 (Nm)/1  "<M_i_b>"
  Demux1/3(z) -> Yawing Moment w.r.t. CG (Nm)/1  "N_ib"
  Demux1/2(y) -> Pitching Moment w.r.t. CG (Nm)/1  "M_ib"
  Demux1/1(x) -> Rolling Moment w.r.t. CG (Nm)/1  "L_ib"
  Demux/3(z) -> Downward Forces (N) (Body Frame)/1  "Z_ib"
  Demux/2(y) -> Lateral Forces (N) (Body Frame)/1  "Y_ib"
  Demux/1(x) -> Forward Forces (N) (Body Frame)/1  "X_ib"
  Bus Selector/2 -> Demux1/1(xyz)  "<Q_i_b>"
  Bus Selector/1 -> Demux/1(xyz)  "<R_i_b>"
  forceLocBus/1 -> Bus Selector/1

== system sim_config2a/Scopes/Aerodynamics/Horizontal Tailplane/Aerodynamics/Local Inflow ==
  localInflowBus : Inport
  Bus Selector : BusSelector  OutputSignals=V_25
  Demux : MATLAB Function  TreatAsAtomicUnit=on
  Downward Velocities (m/s) (Body Frame) : Scope
  Forward Velocities (m/s) (Body Frame) : Scope
  Lateral Velocities (m/s) (Body Frame) : Scope
  wires:
  Demux/3(z) -> Downward Velocities (m/s) (Body Frame)/1  "w_ib"
  Demux/2(y) -> Lateral Velocities (m/s) (Body Frame)/1  "v_ib"
  Demux/1(x) -> Forward Velocities (m/s) (Body Frame)/1  "u_ib"
  Bus Selector/1 -> Demux/1(xyz)  "<V_25>"
  localInflowBus/1 -> Bus Selector/1

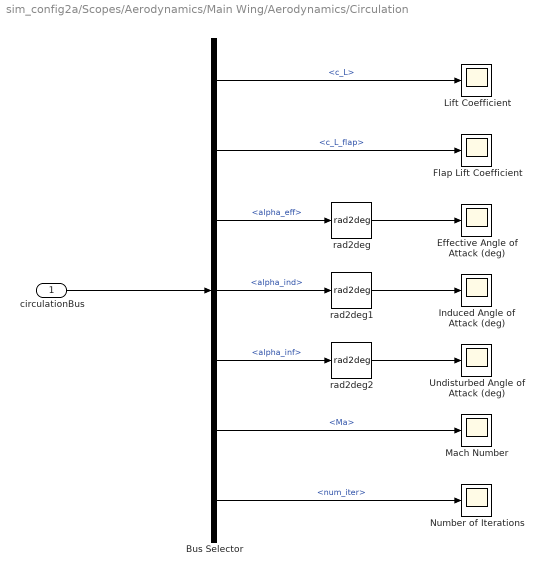
== system sim_config2a/Scopes/Aerodynamics/Main Wing/Aerodynamics/Circulation ==
  circulationBus : Inport
  Bus Selector : BusSelector  OutputSignals=c_L,c_L_flap,alpha_eff,alpha_ind,alpha_inf,Ma,num_iter
  Effective Angle of Attack (deg) : Scope
  Flap Lift Coefficient : Scope
  Induced Angle of Attack (deg) : Scope
  Lift Coefficient : Scope
  Mach Number : Scope
  Number of Iterations : Scope
  Undisturbed Angle of Attack (deg) : Scope
  rad2deg : unit_conversions_lib/rad2deg
      settings: SourceProductName=LADAC
  rad2deg1 : unit_conversions_lib/rad2deg
      settings: SourceProductName=LADAC
  rad2deg2 : unit_conversions_lib/rad2deg
      settings: SourceProductName=LADAC
  wires:
  circulationBus/1 -> Bus Selector/1
  Bus Selector/1 -> Lift Coefficient/1  "<c_L>"
  Bus Selector/2 -> Flap Lift Coefficient/1  "<c_L_flap>"
  Bus Selector/3 -> rad2deg/1  "<alpha_eff>"
  rad2deg/1 -> Effective Angle of Attack (deg)/1
  Bus Selector/4 -> rad2deg1/1  "<alpha_ind>"
  rad2deg1/1 -> Induced Angle of Attack (deg)/1
  Bus Selector/5 -> rad2deg2/1  "<alpha_inf>"
  rad2deg2/1 -> Undisturbed Angle of Attack (deg)/1
  Bus Selector/6 -> Mach Number/1  "<Ma>"
  Bus Selector/7 -> Number of Iterations/1  "<num_iter>"

== system sim_config2a/Scopes/Aerodynamics/Main Wing/Aerodynamics/Global Coefficients ==
  coeffGlobBus : Inport
  Bus Selector : BusSelector  OutputSignals=C_XYZ_b,C_lmn_b
  Force Coefficients (Body Frame) : Scope
  Moment Coefficients (Body Frame) : Scope
  wires:
  coeffGlobBus/1 -> Bus Selector/1
  Bus Selector/1 -> Force Coefficients (Body Frame)/1  "<C_XYZ_b>"
  Bus Selector/2 -> Moment Coefficients (Body Frame)/1  "<C_lmn_b>"

== system sim_config2a/Scopes/Aerodynamics/Main Wing/Aerodynamics/Global Forces ==
  forceGlobBus : Inport
  Bus Selector : BusSelector  OutputSignals=R_b,Q_origin_b
  Force Vector (N) (Body Frame) : Scope
  Moment Vector w.r.t. CG (N) (Body Frame) : Scope
  wires:
  forceGlobBus/1 -> Bus Selector/1
  Bus Selector/1 -> Force Vector (N) (Body Frame)/1  "<R_b>"
  Bus Selector/2 -> Moment Vector w.r.t. CG (N) (Body Frame)/1  "<Q_origin_b>"

== system sim_config2a/Scopes/Aerodynamics/Main Wing/Aerodynamics/Local Coefficients ==
  coeffLocBus : Inport
  Bus Selector : BusSelector  OutputSignals=c_XYZ_b,c_m_airfoil
  Demux : MATLAB Function  TreatAsAtomicUnit=on
  Downward Force Coefficient (Body Frame) : Scope
  Forward Force Coefficient (Body Frame) : Scope
  Lateral Force Coefficient (Body Frame) : Scope
  Pitching Moment Coefficient (c/4) : Scope
  wires:
  coeffLocBus/1 -> Bus Selector/1
  Bus Selector/1 -> Demux/1(xyz)  "<c_XYZ_b>"
  Demux/1(x) -> Forward Force Coefficient (Body Frame)/1  "c_Xb"
  Demux/2(y) -> Lateral Force Coefficient (Body Frame)/1  "c_Yb"
  Demux/3(z) -> Downward Force Coefficient (Body Frame)/1  "c_Zb"
  Bus Selector/2 -> Pitching Moment Coefficient (c/4)/1  "<c_m_airfoil>"

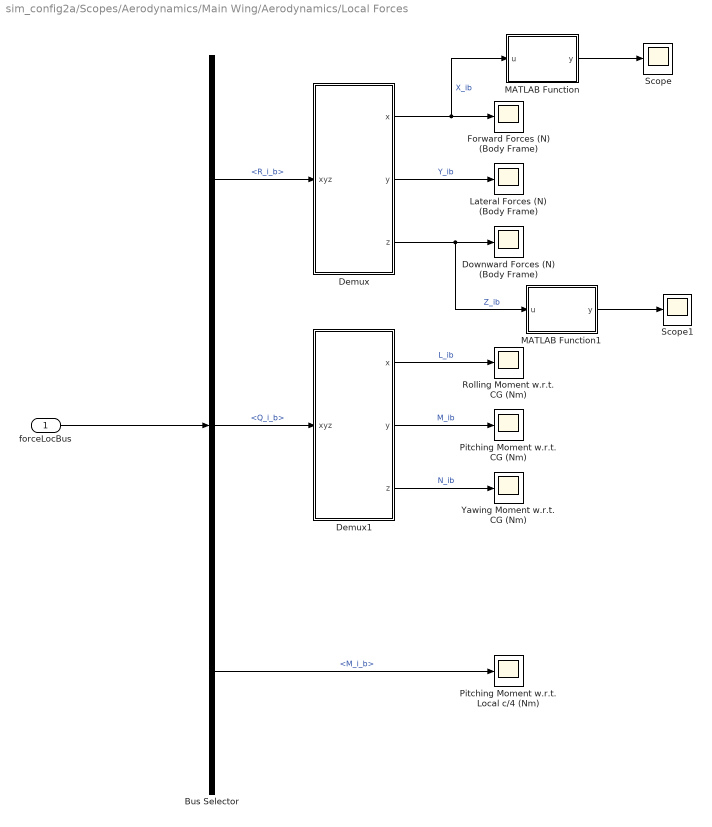
== system sim_config2a/Scopes/Aerodynamics/Main Wing/Aerodynamics/Local Forces ==
  forceLocBus : Inport
  Bus Selector : BusSelector  OutputSignals=R_i_b,Q_i_b,M_i_b
  Demux : MATLAB Function  TreatAsAtomicUnit=on
  Demux1 : MATLAB Function  TreatAsAtomicUnit=on
  Downward Forces (N) (Body Frame) : Scope
  Forward Forces (N) (Body Frame) : Scope
  Lateral Forces (N) (Body Frame) : Scope
  MATLAB Function : MATLAB Function  TreatAsAtomicUnit=on
  MATLAB Function1 : MATLAB Function  TreatAsAtomicUnit=on
  Pitching Moment w.r.t. CG (Nm) : Scope
  Pitching Moment w.r.t. Local c/4 (Nm) : Scope
  Rolling Moment w.r.t. CG (Nm) : Scope
  Scope : Scope
  Scope1 : Scope
  Yawing Moment w.r.t. CG (Nm) : Scope
  wires:
  forceLocBus/1 -> Bus Selector/1
  Bus Selector/1 -> Demux/1(xyz)  "<R_i_b>"
  Bus Selector/2 -> Demux1/1(xyz)  "<Q_i_b>"
  Demux/1(x) -> MATLAB Function/1(u), Forward Forces (N) (Body Frame)/1  "X_ib"
  Demux/2(y) -> Lateral Forces (N) (Body Frame)/1  "Y_ib"
  Demux/3(z) -> MATLAB Function1/1(u), Downward Forces (N) (Body Frame)/1  "Z_ib"
  Demux1/1(x) -> Rolling Moment w.r.t. CG (Nm)/1  "L_ib"
  Demux1/2(y) -> Pitching Moment w.r.t. CG (Nm)/1  "M_ib"
  Demux1/3(z) -> Yawing Moment w.r.t. CG (Nm)/1  "N_ib"
  Bus Selector/3 -> Pitching Moment w.r.t. Local c/4 (Nm)/1  "<M_i_b>"
  MATLAB Function/1(y) -> Scope/1
  MATLAB Function1/1(y) -> Scope1/1

== system sim_config2a/Scopes/Aerodynamics/Main Wing/Aerodynamics/Local Inflow ==
  localInflowBus : Inport
  Bus Selector : BusSelector  OutputSignals=V_25
  Demux : MATLAB Function  TreatAsAtomicUnit=on
  Downward Velocities (m/s) (Body Frame) : Scope
  Forward Velocities (m/s) (Body Frame) : Scope
  Lateral Velocities (m/s) (Body Frame) : Scope
  wires:
  localInflowBus/1 -> Bus Selector/1
  Bus Selector/1 -> Demux/1(xyz)  "<V_25>"
  Demux/1(x) -> Forward Velocities (m/s) (Body Frame)/1  "u_ib"
  Demux/2(y) -> Lateral Velocities (m/s) (Body Frame)/1  "v_ib"
  Demux/3(z) -> Downward Velocities (m/s) (Body Frame)/1  "w_ib"

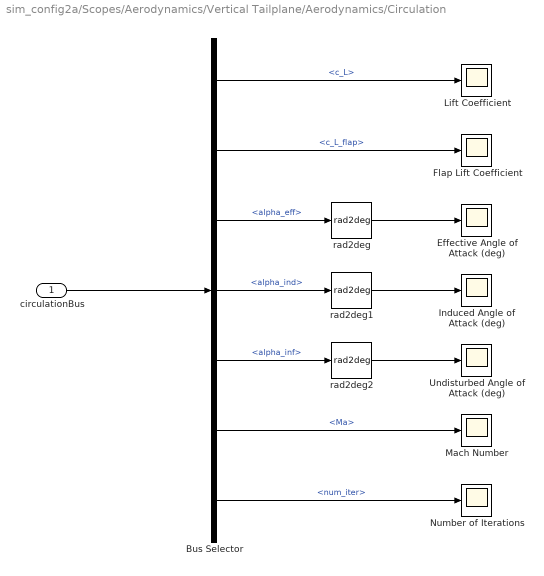
== system sim_config2a/Scopes/Aerodynamics/Vertical Tailplane/Aerodynamics/Circulation ==
  circulationBus : Inport
  Bus Selector : BusSelector  OutputSignals=c_L,c_L_flap,alpha_eff,alpha_ind,alpha_inf,Ma,num_iter
  Effective Angle of Attack (deg) : Scope
  Flap Lift Coefficient : Scope
  Induced Angle of Attack (deg) : Scope
  Lift Coefficient : Scope
  Mach Number : Scope
  Number of Iterations : Scope
  Undisturbed Angle of Attack (deg) : Scope
  rad2deg : unit_conversions_lib/rad2deg
      settings: SourceProductName=LADAC
  rad2deg1 : unit_conversions_lib/rad2deg
      settings: SourceProductName=LADAC
  rad2deg2 : unit_conversions_lib/rad2deg
      settings: SourceProductName=LADAC
  wires:
  circulationBus/1 -> Bus Selector/1
  Bus Selector/1 -> Lift Coefficient/1  "<c_L>"
  Bus Selector/2 -> Flap Lift Coefficient/1  "<c_L_flap>"
  Bus Selector/3 -> rad2deg/1  "<alpha_eff>"
  rad2deg/1 -> Effective Angle of Attack (deg)/1
  Bus Selector/4 -> rad2deg1/1  "<alpha_ind>"
  rad2deg1/1 -> Induced Angle of Attack (deg)/1
  Bus Selector/5 -> rad2deg2/1  "<alpha_inf>"
  rad2deg2/1 -> Undisturbed Angle of Attack (deg)/1
  Bus Selector/6 -> Mach Number/1  "<Ma>"
  Bus Selector/7 -> Number of Iterations/1  "<num_iter>"

== system sim_config2a/Scopes/Aerodynamics/Vertical Tailplane/Aerodynamics/Global Coefficients ==
  coeffGlobBus : Inport
  Bus Selector : BusSelector  OutputSignals=C_XYZ_b,C_lmn_b
  Force Coefficients (Body Frame) : Scope
  Moment Coefficients (Body Frame) : Scope
  wires:
  coeffGlobBus/1 -> Bus Selector/1
  Bus Selector/1 -> Force Coefficients (Body Frame)/1  "<C_XYZ_b>"
  Bus Selector/2 -> Moment Coefficients (Body Frame)/1  "<C_lmn_b>"

== system sim_config2a/Scopes/Aerodynamics/Vertical Tailplane/Aerodynamics/Global Forces ==
  forceGlobBus : Inport
  Bus Selector : BusSelector  OutputSignals=R_b,Q_origin_b
  Force Vector (N) (Body Frame) : Scope
  Moment Vector w.r.t. CG (N) (Body Frame) : Scope
  wires:
  forceGlobBus/1 -> Bus Selector/1
  Bus Selector/1 -> Force Vector (N) (Body Frame)/1  "<R_b>"
  Bus Selector/2 -> Moment Vector w.r.t. CG (N) (Body Frame)/1  "<Q_origin_b>"

== system sim_config2a/Scopes/Aerodynamics/Vertical Tailplane/Aerodynamics/Local Coefficients ==
  coeffLocBus : Inport
  Bus Selector : BusSelector  OutputSignals=c_XYZ_b,c_m_airfoil
  Demux : MATLAB Function  TreatAsAtomicUnit=on
  Downward Force Coefficient (Body Frame) : Scope
  Forward Force Coefficient (Body Frame) : Scope
  Lateral Force Coefficient (Body Frame) : Scope
  Pitching Moment Coefficient (c/4) : Scope
  wires:
  coeffLocBus/1 -> Bus Selector/1
  Bus Selector/1 -> Demux/1(xyz)  "<c_XYZ_b>"
  Demux/1(x) -> Forward Force Coefficient (Body Frame)/1  "c_Xb"
  Demux/2(y) -> Lateral Force Coefficient (Body Frame)/1  "c_Yb"
  Demux/3(z) -> Downward Force Coefficient (Body Frame)/1  "c_Zb"
  Bus Selector/2 -> Pitching Moment Coefficient (c/4)/1  "<c_m_airfoil>"

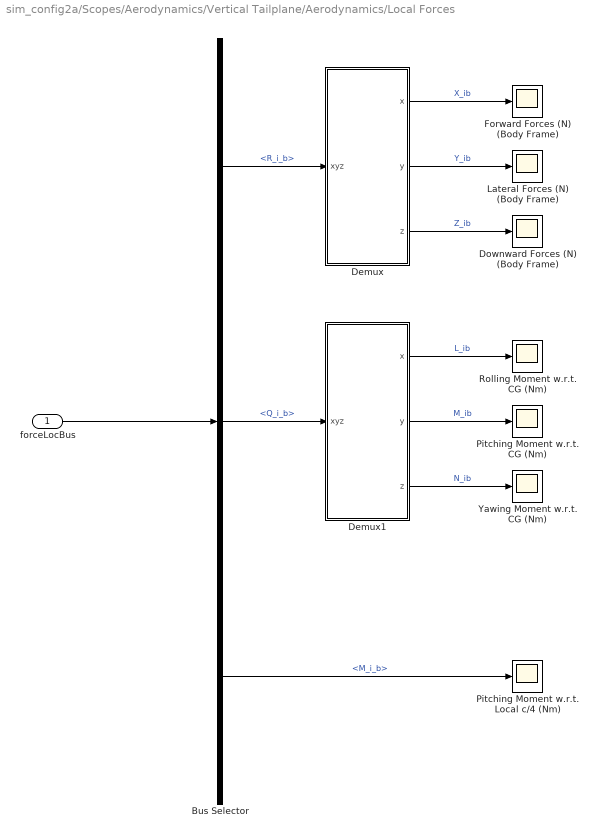
== system sim_config2a/Scopes/Aerodynamics/Vertical Tailplane/Aerodynamics/Local Forces ==
  forceLocBus : Inport
  Bus Selector : BusSelector  OutputSignals=R_i_b,Q_i_b,M_i_b
  Demux : MATLAB Function  TreatAsAtomicUnit=on
  Demux1 : MATLAB Function  TreatAsAtomicUnit=on
  Downward Forces (N) (Body Frame) : Scope
  Forward Forces (N) (Body Frame) : Scope
  Lateral Forces (N) (Body Frame) : Scope
  Pitching Moment w.r.t. CG (Nm) : Scope
  Pitching Moment w.r.t. Local c/4 (Nm) : Scope
  Rolling Moment w.r.t. CG (Nm) : Scope
  Yawing Moment w.r.t. CG (Nm) : Scope
  wires:
  forceLocBus/1 -> Bus Selector/1
  Bus Selector/1 -> Demux/1(xyz)  "<R_i_b>"
  Bus Selector/2 -> Demux1/1(xyz)  "<Q_i_b>"
  Demux/1(x) -> Forward Forces (N) (Body Frame)/1  "X_ib"
  Demux/2(y) -> Lateral Forces (N) (Body Frame)/1  "Y_ib"
  Demux/3(z) -> Downward Forces (N) (Body Frame)/1  "Z_ib"
  Demux1/1(x) -> Rolling Moment w.r.t. CG (Nm)/1  "L_ib"
  Demux1/2(y) -> Pitching Moment w.r.t. CG (Nm)/1  "M_ib"
  Demux1/3(z) -> Yawing Moment w.r.t. CG (Nm)/1  "N_ib"
  Bus Selector/3 -> Pitching Moment w.r.t. Local c/4 (Nm)/1  "<M_i_b>"

== system sim_config2a/Scopes/Aerodynamics/Vertical Tailplane/Aerodynamics/Local Inflow ==
  localInflowBus : Inport
  Bus Selector : BusSelector  OutputSignals=V_25
  Demux : MATLAB Function  TreatAsAtomicUnit=on
  Downward Velocities (m/s) (Body Frame) : Scope
  Forward Velocities (m/s) (Body Frame) : Scope
  Lateral Velocities (m/s) (Body Frame) : Scope
  wires:
  localInflowBus/1 -> Bus Selector/1
  Bus Selector/1 -> Demux/1(xyz)  "<V_25>"
  Demux/1(x) -> Forward Velocities (m/s) (Body Frame)/1  "u_ib"
  Demux/2(y) -> Lateral Velocities (m/s) (Body Frame)/1  "v_ib"
  Demux/3(z) -> Downward Velocities (m/s) (Body Frame)/1  "w_ib"

== matlab function sim_config2a/Scopes/Aerodynamics/Vertical Tailplane/Aerodynamics/Local Coefficients/Demux ==
  data: x output; xyz input; y output; z output
function [x,y,z] = fcn(xyz)
x = xyz(1,:);
y = xyz(2,:);
z = xyz(3,:);
end

== matlab function sim_config2a/Scopes/Aerodynamics/Main Wing/Aerodynamics/Local Forces/Demux ==
  data: x output; xyz input; y output; z output
function [x,y,z] = fcn(xyz)
x = xyz(1,:);
y = xyz(2,:);
z = xyz(3,:);
end

== matlab function sim_config2a/Scopes/Aerodynamics/Vertical Tailplane/Aerodynamics/Local Forces/Demux ==
  data: x output; xyz input; y output; z output
function [x,y,z] = fcn(xyz)
x = xyz(1,:);
y = xyz(2,:);
z = xyz(3,:);
end

== matlab function sim_config2a/Scopes/Aerodynamics/Vertical Tailplane/Aerodynamics/Local Forces/Demux1 ==
  data: x output; xyz input; y output; z output
function [x,y,z] = fcn(xyz)
x = xyz(1,:);
y = xyz(2,:);
z = xyz(3,:);
end

== matlab function sim_config2a/Scopes/Aerodynamics/Vertical Tailplane/Aerodynamics/Local Inflow/Demux ==
  data: x output; xyz input; y output; z output
function [x,y,z] = fcn(xyz)
x = xyz(1,:);
y = xyz(2,:);
z = xyz(3,:);
end

== matlab function sim_config2a/Scopes/Aerodynamics/Vertical Tailplane/Wind//Slipstream/Demux ==
  data: x output; xyz input; y output; z output
function [x,y,z] = fcn(xyz)
x = xyz(1,:);
y = xyz(2,:);
z = xyz(3,:);
end

== matlab function sim_config2a/Scopes/Aerodynamics/Main Wing/Aerodynamics/Local Forces/MATLAB Function ==
  data: u input; y output
function y = fcn(u)

y = u([1:10,end-9:end]);

== matlab function sim_config2a/Scopes/Aerodynamics/Main Wing/Aerodynamics/Local Forces/MATLAB Function1 ==
  data: u input; y output
function y = fcn(u)

y = u([1:10,end-9:end]);

== matlab function sim_config2a/MATLAB Function ==
  data: cmd input; ai_l output; ai_r output; el output; ru output; thr output
function [ai_l,ai_r,el,ru,thr] = fcn(cmd)
ai_l = cmd(1);
ai_r = cmd(2);
el = cmd(3);
ru = cmd(4);
thr = cmd(5:end);
end

== matlab function sim_config2a/Trim Cmd/u0 to Cmd ==
  data: u0 input; cmd output; num_props parameter
function cmd = fcn(u0,num_props)
cmd = [u0(1:end-1);repmat(u0(end),num_props,1)];
end

== matlab function sim_config2a/Send to FlightGear/Flight Gear Animation (plane)/MATLAB Function ==
  data: u input; y output; y2 output; y3 output
function [y,y2,y3] = fcn(u)

y = u(1:4);
y2 = u(5:8);
y3 = zeros(4,1);
y3(1:2) = u(9:10);

== matlab function sim_config2a/Send to FlightGear/MATLAB Function ==
  data: u input; y output
function y = fcn(u)

y = u([1,end]);

== matlab function sim_config2a/Send to FlightGear/UmrechnungDeg ==
  data: u input; y output
function y = fcn(u)

y = rad2deg(u)+54.7;

== matlab function sim_config2a/Scopes/Aerodynamics/Main Wing/Aerodynamics/Local Coefficients/Demux ==
  data: x output; xyz input; y output; z output
function [x,y,z] = fcn(xyz)
x = xyz(1,:);
y = xyz(2,:);
z = xyz(3,:);
end

== matlab function sim_config2a/Scopes/Aerodynamics/Main Wing/Aerodynamics/Local Forces/Demux1 ==
  data: x output; xyz input; y output; z output
function [x,y,z] = fcn(xyz)
x = xyz(1,:);
y = xyz(2,:);
z = xyz(3,:);
end

== matlab function sim_config2a/Scopes/Aerodynamics/Main Wing/Aerodynamics/Local Inflow/Demux ==
  data: x output; xyz input; y output; z output
function [x,y,z] = fcn(xyz)
x = xyz(1,:);
y = xyz(2,:);
z = xyz(3,:);
end

== matlab function sim_config2a/Scopes/Aerodynamics/Main Wing/Wind//Slipstream/Demux ==
  data: x output; xyz input; y output; z output
function [x,y,z] = fcn(xyz)
x = xyz(1,:);
y = xyz(2,:);
z = xyz(3,:);
end

== matlab function sim_config2a/Scopes/Aerodynamics/Horizontal Tailplane/Aerodynamics/Local Coefficients/Demux ==
  data: x output; xyz input; y output; z output
function [x,y,z] = fcn(xyz)
x = xyz(1,:);
y = xyz(2,:);
z = xyz(3,:);
end

== matlab function sim_config2a/Scopes/Aerodynamics/Horizontal Tailplane/Aerodynamics/Local Forces/Demux ==
  data: x output; xyz input; y output; z output
function [x,y,z] = fcn(xyz)
x = xyz(1,:);
y = xyz(2,:);
z = xyz(3,:);
end

== matlab function sim_config2a/Scopes/Aerodynamics/Horizontal Tailplane/Aerodynamics/Local Forces/Demux1 ==
  data: x output; xyz input; y output; z output
function [x,y,z] = fcn(xyz)
x = xyz(1,:);
y = xyz(2,:);
z = xyz(3,:);
end

== matlab function sim_config2a/Scopes/Aerodynamics/Horizontal Tailplane/Aerodynamics/Local Inflow/Demux ==
  data: x output; xyz input; y output; z output
function [x,y,z] = fcn(xyz)
x = xyz(1,:);
y = xyz(2,:);
z = xyz(3,:);
end

== matlab function sim_config2a/Scopes/Aerodynamics/Horizontal Tailplane/Wind//Slipstream/Demux ==
  data: x output; xyz input; y output; z output
function [x,y,z] = fcn(xyz)
x = xyz(1,:);
y = xyz(2,:);
z = xyz(3,:);
end
